simulink model "superposition"  (R2025b)
settings: Solver=VariableStepAuto  StartTime=0.0  StopTime=60  RelTol=1e-3
values from neighbouring files (symbols this model uses):
  A = [0 1 ... (first row only)    [esercitazione3.m]
  B = [0 ... (first row only)    [esercitazione3.m]
  C = [1 0]    [esercitazione3.m]
  D = 0    [esercitazione3.m]
  step_amplitude1 = 0.1    [esercitazione3.m]
  step_amplitude2 = 0.05    [esercitazione3.m]
  x0 = [0;0]    [esercitazione3.m]    (also in s_func.m = [0 0]')
settings Model: Creator=papidrago  LastModifiedBy=papidrago

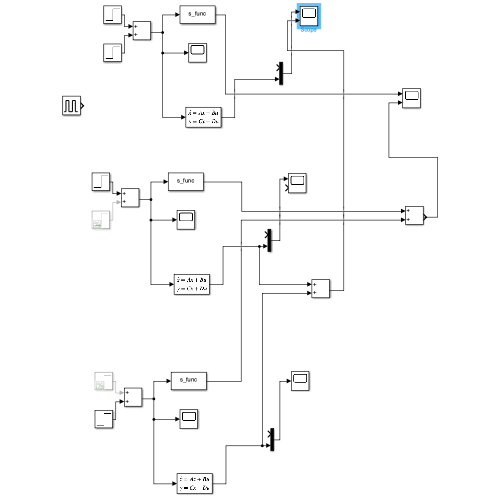
[thumbnail: Simulink's stored preview of the top-level diagram]
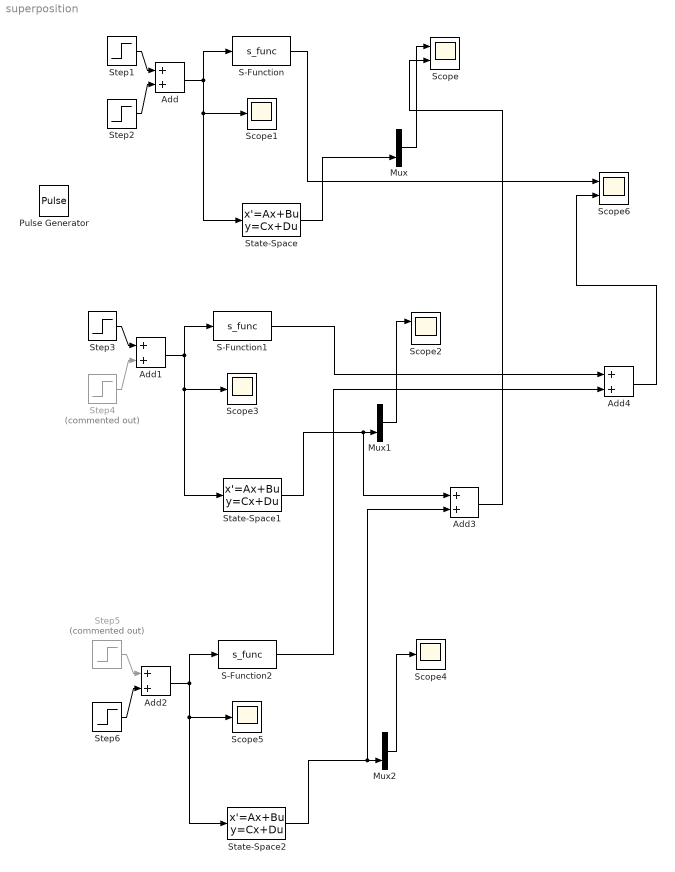
== system superposition ==
  Add{,1..4} (5 alike) : Sum
  Mux : Mux  Inputs=2
  Mux1 : Mux  Inputs=2
  Mux2 : Mux  Inputs=2
  Pulse Generator : DiscretePulseGenerator  PulseType=Time based  Period=10  PulseWidth=5
  S-Function : S-Function  FunctionName=s_func  Parameters=x0, m, h, k  SFunctionDeploymentMode=off  EnableBusSupport=off
  S-Function1 : S-Function  FunctionName=s_func  Parameters=x0, m, h, k  SFunctionDeploymentMode=off  EnableBusSupport=off
  S-Function2 : S-Function  FunctionName=s_func  Parameters=x0, m, h, k  SFunctionDeploymentMode=off  EnableBusSupport=off
  Scope : Scope  NumInputPorts=2
      settings: ActiveDisplayYMinimum=-0.062315649594024386  ActiveDisplayYMaximum=0.56084084634621956
  Scope{1,3..5} (4 alike) : Scope
      Scope1 settings: ActiveDisplayYMinimum=0.13702714836078106  ActiveDisplayYMaximum=0.42488289609569052
      Scope3 settings: ActiveDisplayYMinimum=0.13702714836078106  ActiveDisplayYMaximum=0.42488289609569052  DataLoggingVariableName=ScopeData3
      Scope4 settings: ActiveDisplayYMinimum=-0.062315649594024386  ActiveDisplayYMaximum=0.56084084634621956  DataLoggingVariableName=ScopeData4
      Scope5 settings: ActiveDisplayYMinimum=0.13702714836078106  ActiveDisplayYMaximum=0.42488289609569052  DataLoggingVariableName=ScopeData5
  Scope2 : Scope  NumInputPorts=2
      settings: ActiveDisplayYMinimum=-0.062315649594024386  ActiveDisplayYMaximum=0.56084084634621956  DataLoggingVariableName=ScopeData2
  Scope6 : Scope  NumInputPorts=2
      settings: ActiveDisplayYMinimum=-0.31167313097119548  ActiveDisplayYMaximum=2.80505817874076  DataLoggingVariableName=ScopeData6
  State-Space : StateSpace  A=A  B=B  C=C  D=D  InitialCondition=x0
  State-Space1 : StateSpace  A=A  B=B  C=C  D=D  InitialCondition=x0
  State-Space2 : StateSpace  A=A  B=B  C=C  D=D  InitialCondition=x0
  Step1 : Step  After=step_amplitude1  SampleTime=0
  Step2 : Step  After=step_amplitude2  SampleTime=0
  Step3 : Step  After=step_amplitude1  SampleTime=0
  Step4 : Step  Commented=on  After=step_amplitude2  SampleTime=0
  Step5 : Step  Commented=on  After=step_amplitude1  SampleTime=0
  Step6 : Step  After=step_amplitude2  SampleTime=0
  wires:
  Step2/1 -> Add/2
  Step1/1 -> Add/1
  Add/1 -> Scope1/1, State-Space/1, S-Function/1
  State-Space/1 -> Mux/2
  Mux/1 -> Scope/1
  Step3/1 -> Add1/1
  Step4/1 -> Add1/2
  Mux1/1 -> Scope2/1
  Add1/1 -> Scope3/1, State-Space1/1, S-Function1/1
  State-Space1/1 -> Add3/1, Mux1/2
  Step5/1 -> Add2/1
  Add2/1 -> Scope5/1, State-Space2/1, S-Function2/1
  State-Space2/1 -> Add3/2, Mux2/2
  Mux2/1 -> Scope4/1
  Step6/1 -> Add2/2
  Add3/1 -> Scope/2
  S-Function/1 -> Scope6/1
  S-Function1/1 -> Add4/1
  S-Function2/1 -> Add4/2
  Add4/1 -> Scope6/2
